simulink model "adc_5g_e2v"  (R2018a)
settings: Solver=VariableStepAuto  StartTime=0.0  StopTime=10.0  RelTol=1e-3
libraries: xbsIndex_r4 x68
settings Model: Creator=jkocz  LastModifiedBy=jackh
settings CodeAppCC: StateflowObjectComments=on

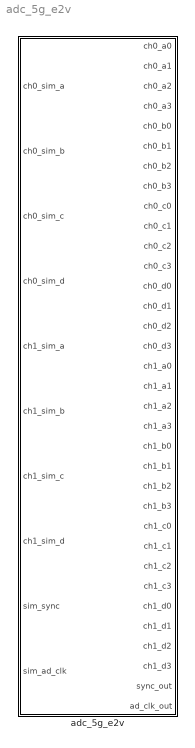
== system adc_5g_e2v ==
  adc_5g_e2v : Subsystem  Tag=xps:adc_5g_e2v  mask(E2V_5g_adc){adc_mode=4-Channel, output_mode=normal mode, chips_num=2, adc_loc=FMC1, f_sample=1000}
      mask prompts: adc_mode "ADC Work mode"; output_mode "ADC Output mode"; chips_num "Number of ADC chips"; adc_loc "ADC board location"; f_sample "ADC Clock Rate(Mhz)"
      mask init:
      | adc_5g_e2v_init(gcb,...
      |     'adc_mode', adc_mode,...
      |     'chips_num',chips_num,...
      |     'adc_loc',adc_loc,...
      |     'f_sample',f_sample);
      mask TypeOptions adc_mode: 1-Channel | 2-Channel | 4-Channel
      mask TypeOptions output_mode: normal mode | test mode
      mask TypeOptions chips_num: 1 | 2
      mask TypeOptions adc_loc: FMC1 | FMC2

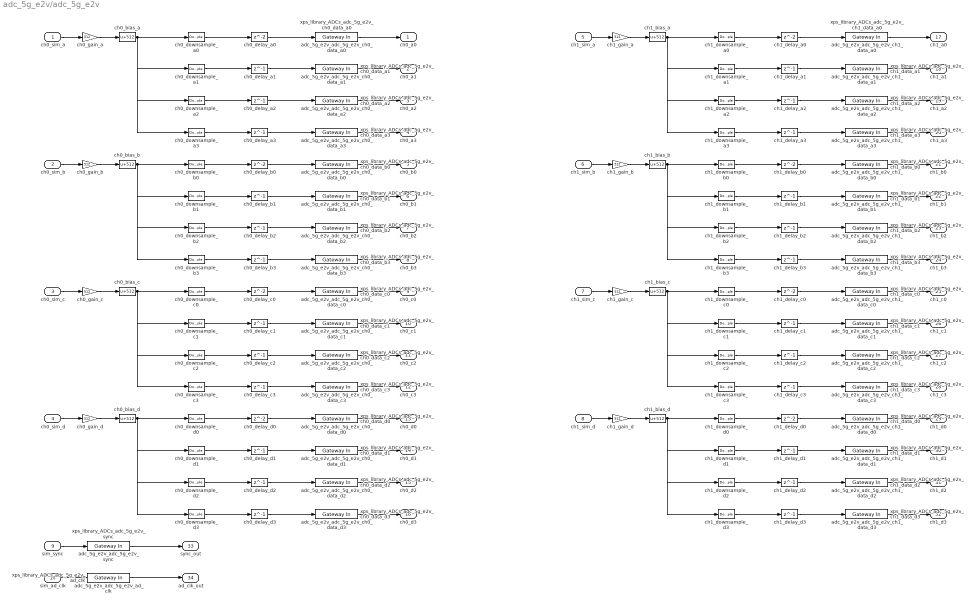
== system adc_5g_e2v/adc_5g_e2v ==
  ch0_sim_a : Inport
  ch0_sim_b : Inport  Port=2
  ch0_sim_c : Inport  Port=3
  ch0_sim_d : Inport  Port=4
  ch1_sim_a : Inport  Port=5
  ch1_sim_b : Inport  Port=6
  ch1_sim_c : Inport  Port=7
  ch1_sim_d : Inport  Port=8
  sim_sync : Inport  Port=9
  sim_ad_clk : Inport  Port=10
  adc_5g_e2v_adc_5g_e2v_ad_clk : xbsIndex_r4/Gateway In  gui_display_data_type=Fixed-point  arith_type=Boolean  n_bits=16  bin_pt=14  preci_type=Single  exp_width=8  frac_width=24  rows=1  columns=1  quantization="Round  (unbiased: +/- Inf)"  overflow=Saturate  period=1  UseAsADC=off  ADCChannel='1'  interface=None  automatic_assignment=on  address_offset=hex2dec('00')  intf_name=''  intf_description=''  default_value=0  timing_constraint=None  locs_specified=off  LOCs={}  io_standard={}  inherit_from_input=off  hdl_port=on  dbl_ovrd=off  block_type=gatewayin
  adc_5g_e2v_adc_5g_e2v_ch0_data_a{0..3} (4 alike) : xbsIndex_r4/Gateway In  gui_display_data_type=Fixed-point  arith_type=Unsigned  n_bits=10  bin_pt=0  preci_type=Single  exp_width=8  frac_width=24  rows=1  columns=1  quantization=Truncate  overflow=Wrap  period=1  UseAsADC=off  ADCChannel='1'  interface=None  automatic_assignment=on  address_offset=hex2dec('00')  intf_name=''  intf_description=''  default_value=0  timing_constraint=None  locs_specified=off  LOCs={}  io_standard={}  inherit_from_input=off  hdl_port=on  dbl_ovrd=off  block_type=gatewayin
  adc_5g_e2v_adc_5g_e2v_ch0_data_b{0..3} (4 alike) : xbsIndex_r4/Gateway In  gui_display_data_type=Fixed-point  arith_type=Unsigned  n_bits=10  bin_pt=0  preci_type=Single  exp_width=8  frac_width=24  rows=1  columns=1  quantization=Truncate  overflow=Wrap  period=1  UseAsADC=off  ADCChannel='1'  interface=None  automatic_assignment=on  address_offset=hex2dec('00')  intf_name=''  intf_description=''  default_value=0  timing_constraint=None  locs_specified=off  LOCs={}  io_standard={}  inherit_from_input=off  hdl_port=on  dbl_ovrd=off  block_type=gatewayin
  adc_5g_e2v_adc_5g_e2v_ch0_data_c{0..3} (4 alike) : xbsIndex_r4/Gateway In  gui_display_data_type=Fixed-point  arith_type=Unsigned  n_bits=10  bin_pt=0  preci_type=Single  exp_width=8  frac_width=24  rows=1  columns=1  quantization=Truncate  overflow=Wrap  period=1  UseAsADC=off  ADCChannel='1'  interface=None  automatic_assignment=on  address_offset=hex2dec('00')  intf_name=''  intf_description=''  default_value=0  timing_constraint=None  locs_specified=off  LOCs={}  io_standard={}  inherit_from_input=off  hdl_port=on  dbl_ovrd=off  block_type=gatewayin
  adc_5g_e2v_adc_5g_e2v_ch0_data_d{0..3} (4 alike) : xbsIndex_r4/Gateway In  gui_display_data_type=Fixed-point  arith_type=Unsigned  n_bits=10  bin_pt=0  preci_type=Single  exp_width=8  frac_width=24  rows=1  columns=1  quantization=Truncate  overflow=Wrap  period=1  UseAsADC=off  ADCChannel='1'  interface=None  automatic_assignment=on  address_offset=hex2dec('00')  intf_name=''  intf_description=''  default_value=0  timing_constraint=None  locs_specified=off  LOCs={}  io_standard={}  inherit_from_input=off  hdl_port=on  dbl_ovrd=off  block_type=gatewayin
  adc_5g_e2v_adc_5g_e2v_ch1_data_a{0..3} (4 alike) : xbsIndex_r4/Gateway In  gui_display_data_type=Fixed-point  arith_type=Unsigned  n_bits=10  bin_pt=0  preci_type=Single  exp_width=8  frac_width=24  rows=1  columns=1  quantization=Truncate  overflow=Wrap  period=1  UseAsADC=off  ADCChannel='1'  interface=None  automatic_assignment=on  address_offset=hex2dec('00')  intf_name=''  intf_description=''  default_value=0  timing_constraint=None  locs_specified=off  LOCs={}  io_standard={}  inherit_from_input=off  hdl_port=on  dbl_ovrd=off  block_type=gatewayin
  adc_5g_e2v_adc_5g_e2v_ch1_data_b{0..3} (4 alike) : xbsIndex_r4/Gateway In  gui_display_data_type=Fixed-point  arith_type=Unsigned  n_bits=10  bin_pt=0  preci_type=Single  exp_width=8  frac_width=24  rows=1  columns=1  quantization=Truncate  overflow=Wrap  period=1  UseAsADC=off  ADCChannel='1'  interface=None  automatic_assignment=on  address_offset=hex2dec('00')  intf_name=''  intf_description=''  default_value=0  timing_constraint=None  locs_specified=off  LOCs={}  io_standard={}  inherit_from_input=off  hdl_port=on  dbl_ovrd=off  block_type=gatewayin
  adc_5g_e2v_adc_5g_e2v_ch1_data_c{0..3} (4 alike) : xbsIndex_r4/Gateway In  gui_display_data_type=Fixed-point  arith_type=Unsigned  n_bits=10  bin_pt=0  preci_type=Single  exp_width=8  frac_width=24  rows=1  columns=1  quantization=Truncate  overflow=Wrap  period=1  UseAsADC=off  ADCChannel='1'  interface=None  automatic_assignment=on  address_offset=hex2dec('00')  intf_name=''  intf_description=''  default_value=0  timing_constraint=None  locs_specified=off  LOCs={}  io_standard={}  inherit_from_input=off  hdl_port=on  dbl_ovrd=off  block_type=gatewayin
  adc_5g_e2v_adc_5g_e2v_ch1_data_d{0..3} (4 alike) : xbsIndex_r4/Gateway In  gui_display_data_type=Fixed-point  arith_type=Unsigned  n_bits=10  bin_pt=0  preci_type=Single  exp_width=8  frac_width=24  rows=1  columns=1  quantization=Truncate  overflow=Wrap  period=1  UseAsADC=off  ADCChannel='1'  interface=None  automatic_assignment=on  address_offset=hex2dec('00')  intf_name=''  intf_description=''  default_value=0  timing_constraint=None  locs_specified=off  LOCs={}  io_standard={}  inherit_from_input=off  hdl_port=on  dbl_ovrd=off  block_type=gatewayin
  adc_5g_e2v_adc_5g_e2v_sync : xbsIndex_r4/Gateway In  gui_display_data_type=Fixed-point  arith_type=Boolean  n_bits=16  bin_pt=14  preci_type=Single  exp_width=8  frac_width=24  rows=1  columns=1  quantization="Round  (unbiased: +/- Inf)"  overflow=Saturate  period=1  UseAsADC=off  ADCChannel='1'  interface=None  automatic_assignment=on  address_offset=hex2dec('00')  intf_name=''  intf_description=''  default_value=0  timing_constraint=None  locs_specified=off  LOCs={}  io_standard={}  inherit_from_input=off  hdl_port=on  dbl_ovrd=off  block_type=gatewayin
  ch0_bias_a : Bias  Bias=512  SaturateOnIntegerOverflow=on
  ch0_bias_b : Bias  Bias=512  SaturateOnIntegerOverflow=on
  ch0_bias_c : Bias  Bias=512  SaturateOnIntegerOverflow=on
  ch0_bias_d : Bias  Bias=512  SaturateOnIntegerOverflow=on
  ch0_delay_a0 : Delay  InitialCondition=0  InputProcessing=Inherited
  ch0_delay_a1 : Delay  DelayLength=1  InitialCondition=0  InputProcessing=Inherited
  ch0_delay_a2 : Delay  DelayLength=1  InitialCondition=0  InputProcessing=Inherited
  ch0_delay_a3 : Delay  DelayLength=1  InitialCondition=0  InputProcessing=Inherited
  ch0_delay_b0 : Delay  InitialCondition=0  InputProcessing=Inherited
  ch0_delay_b1 : Delay  DelayLength=1  InitialCondition=0  InputProcessing=Inherited
  ch0_delay_b2 : Delay  DelayLength=1  InitialCondition=0  InputProcessing=Inherited
  ch0_delay_b3 : Delay  DelayLength=1  InitialCondition=0  InputProcessing=Inherited
  ch0_delay_c0 : Delay  InitialCondition=0  InputProcessing=Inherited
  ch0_delay_c1 : Delay  DelayLength=1  InitialCondition=0  InputProcessing=Inherited
  ch0_delay_c2 : Delay  DelayLength=1  InitialCondition=0  InputProcessing=Inherited
  ch0_delay_c3 : Delay  DelayLength=1  InitialCondition=0  InputProcessing=Inherited
  ch0_delay_d0 : Delay  InitialCondition=0  InputProcessing=Inherited
  ch0_delay_d1 : Delay  DelayLength=1  InitialCondition=0  InputProcessing=Inherited
  ch0_delay_d2 : Delay  DelayLength=1  InitialCondition=0  InputProcessing=Inherited
  ch0_delay_d3 : Delay  DelayLength=1  InitialCondition=0  InputProcessing=Inherited
  ch0_downsample_a0 : DownSample  N=4  RateOptions=Allow multirate processing
  ch0_downsample_a1 : DownSample  N=4  phase=1  RateOptions=Allow multirate processing
  ch0_downsample_a2 : DownSample  N=4  phase=2  RateOptions=Allow multirate processing
  ch0_downsample_a3 : DownSample  N=4  phase=3  RateOptions=Allow multirate processing
  ch0_downsample_b0 : DownSample  N=4  RateOptions=Allow multirate processing
  ch0_downsample_b1 : DownSample  N=4  phase=1  RateOptions=Allow multirate processing
  ch0_downsample_b2 : DownSample  N=4  phase=2  RateOptions=Allow multirate processing
  ch0_downsample_b3 : DownSample  N=4  phase=3  RateOptions=Allow multirate processing
  ch0_downsample_c0 : DownSample  N=4  RateOptions=Allow multirate processing
  ch0_downsample_c1 : DownSample  N=4  phase=1  RateOptions=Allow multirate processing
  ch0_downsample_c2 : DownSample  N=4  phase=2  RateOptions=Allow multirate processing
  ch0_downsample_c3 : DownSample  N=4  phase=3  RateOptions=Allow multirate processing
  ch0_downsample_d0 : DownSample  N=4  RateOptions=Allow multirate processing
  ch0_downsample_d1 : DownSample  N=4  phase=1  RateOptions=Allow multirate processing
  ch0_downsample_d2 : DownSample  N=4  phase=2  RateOptions=Allow multirate processing
  ch0_downsample_d3 : DownSample  N=4  phase=3  RateOptions=Allow multirate processing
  ch0_gain_a : Gain  Gain=512  SaturateOnIntegerOverflow=on  OutDataTypeStr=Inherit: Same as input  ParamDataTypeStr=Inherit: Same as input
  ch0_gain_b : Gain  Gain=512  SaturateOnIntegerOverflow=on  OutDataTypeStr=Inherit: Same as input  ParamDataTypeStr=Inherit: Same as input
  ch0_gain_c : Gain  Gain=512  SaturateOnIntegerOverflow=on  OutDataTypeStr=Inherit: Same as input  ParamDataTypeStr=Inherit: Same as input
  ch0_gain_d : Gain  Gain=512  SaturateOnIntegerOverflow=on  OutDataTypeStr=Inherit: Same as input  ParamDataTypeStr=Inherit: Same as input
  ch1_bias_a : Bias  Bias=512  SaturateOnIntegerOverflow=on
  ch1_bias_b : Bias  Bias=512  SaturateOnIntegerOverflow=on
  ch1_bias_c : Bias  Bias=512  SaturateOnIntegerOverflow=on
  ch1_bias_d : Bias  Bias=512  SaturateOnIntegerOverflow=on
  ch1_delay_a0 : Delay  InitialCondition=0  InputProcessing=Inherited
  ch1_delay_a1 : Delay  DelayLength=1  InitialCondition=0  InputProcessing=Inherited
  ch1_delay_a2 : Delay  DelayLength=1  InitialCondition=0  InputProcessing=Inherited
  ch1_delay_a3 : Delay  DelayLength=1  InitialCondition=0  InputProcessing=Inherited
  ch1_delay_b0 : Delay  InitialCondition=0  InputProcessing=Inherited
  ch1_delay_b1 : Delay  DelayLength=1  InitialCondition=0  InputProcessing=Inherited
  ch1_delay_b2 : Delay  DelayLength=1  InitialCondition=0  InputProcessing=Inherited
  ch1_delay_b3 : Delay  DelayLength=1  InitialCondition=0  InputProcessing=Inherited
  ch1_delay_c0 : Delay  InitialCondition=0  InputProcessing=Inherited
  ch1_delay_c1 : Delay  DelayLength=1  InitialCondition=0  InputProcessing=Inherited
  ch1_delay_c2 : Delay  DelayLength=1  InitialCondition=0  InputProcessing=Inherited
  ch1_delay_c3 : Delay  DelayLength=1  InitialCondition=0  InputProcessing=Inherited
  ch1_delay_d0 : Delay  InitialCondition=0  InputProcessing=Inherited
  ch1_delay_d1 : Delay  DelayLength=1  InitialCondition=0  InputProcessing=Inherited
  ch1_delay_d2 : Delay  DelayLength=1  InitialCondition=0  InputProcessing=Inherited
  ch1_delay_d3 : Delay  DelayLength=1  InitialCondition=0  InputProcessing=Inherited
  ch1_downsample_a0 : DownSample  N=4  RateOptions=Allow multirate processing
  ch1_downsample_a1 : DownSample  N=4  phase=1  RateOptions=Allow multirate processing
  ch1_downsample_a2 : DownSample  N=4  phase=2  RateOptions=Allow multirate processing
  ch1_downsample_a3 : DownSample  N=4  phase=3  RateOptions=Allow multirate processing
  ch1_downsample_b0 : DownSample  N=4  RateOptions=Allow multirate processing
  ch1_downsample_b1 : DownSample  N=4  phase=1  RateOptions=Allow multirate processing
  ch1_downsample_b2 : DownSample  N=4  phase=2  RateOptions=Allow multirate processing
  ch1_downsample_b3 : DownSample  N=4  phase=3  RateOptions=Allow multirate processing
  ch1_downsample_c0 : DownSample  N=4  RateOptions=Allow multirate processing
  ch1_downsample_c1 : DownSample  N=4  phase=1  RateOptions=Allow multirate processing
  ch1_downsample_c2 : DownSample  N=4  phase=2  RateOptions=Allow multirate processing
  ch1_downsample_c3 : DownSample  N=4  phase=3  RateOptions=Allow multirate processing
  ch1_downsample_d0 : DownSample  N=4  RateOptions=Allow multirate processing
  ch1_downsample_d1 : DownSample  N=4  phase=1  RateOptions=Allow multirate processing
  ch1_downsample_d2 : DownSample  N=4  phase=2  RateOptions=Allow multirate processing
  ch1_downsample_d3 : DownSample  N=4  phase=3  RateOptions=Allow multirate processing
  ch1_gain_a : Gain  Gain=512  SaturateOnIntegerOverflow=on  OutDataTypeStr=Inherit: Same as input  ParamDataTypeStr=Inherit: Same as input
  ch1_gain_b : Gain  Gain=512  SaturateOnIntegerOverflow=on  OutDataTypeStr=Inherit: Same as input  ParamDataTypeStr=Inherit: Same as input
  ch1_gain_c : Gain  Gain=512  SaturateOnIntegerOverflow=on  OutDataTypeStr=Inherit: Same as input  ParamDataTypeStr=Inherit: Same as input
  ch1_gain_d : Gain  Gain=512  SaturateOnIntegerOverflow=on  OutDataTypeStr=Inherit: Same as input  ParamDataTypeStr=Inherit: Same as input
  xps_library_ADCs_adc_5g_e2v_ad_clk : xbsIndex_r4/Gateway In  gui_display_data_type=Fixed-point  arith_type=Boolean  n_bits=16  bin_pt=14  preci_type=Single  exp_width=8  frac_width=24  rows=1  columns=1  quantization="Round  (unbiased: +/- Inf)"  overflow=Saturate  period=1  UseAsADC=off  ADCChannel='1'  interface=None  automatic_assignment=on  address_offset=hex2dec('00')  intf_name=''  intf_description=''  default_value=0  timing_constraint=None  locs_specified=off  LOCs={}  io_standard={}  inherit_from_input=off  hdl_port=on  dbl_ovrd=off  block_type=gatewayin
  xps_library_ADCs_adc_5g_e2v_ch0_data_a{0..3} (4 alike) : xbsIndex_r4/Gateway In  gui_display_data_type=Fixed-point  arith_type=Unsigned  n_bits=10  bin_pt=0  preci_type=Single  exp_width=8  frac_width=24  rows=1  columns=1  quantization=Truncate  overflow=Wrap  period=1  UseAsADC=off  ADCChannel='1'  interface=None  automatic_assignment=on  address_offset=hex2dec('00')  intf_name=''  intf_description=''  default_value=0  timing_constraint=None  locs_specified=off  LOCs={}  io_standard={}  inherit_from_input=off  hdl_port=on  dbl_ovrd=off  block_type=gatewayin
  xps_library_ADCs_adc_5g_e2v_ch0_data_b{0..3} (4 alike) : xbsIndex_r4/Gateway In  gui_display_data_type=Fixed-point  arith_type=Unsigned  n_bits=10  bin_pt=0  preci_type=Single  exp_width=8  frac_width=24  rows=1  columns=1  quantization=Truncate  overflow=Wrap  period=1  UseAsADC=off  ADCChannel='1'  interface=None  automatic_assignment=on  address_offset=hex2dec('00')  intf_name=''  intf_description=''  default_value=0  timing_constraint=None  locs_specified=off  LOCs={}  io_standard={}  inherit_from_input=off  hdl_port=on  dbl_ovrd=off  block_type=gatewayin
  xps_library_ADCs_adc_5g_e2v_ch0_data_c{0..3} (4 alike) : xbsIndex_r4/Gateway In  gui_display_data_type=Fixed-point  arith_type=Unsigned  n_bits=10  bin_pt=0  preci_type=Single  exp_width=8  frac_width=24  rows=1  columns=1  quantization=Truncate  overflow=Wrap  period=1  UseAsADC=off  ADCChannel='1'  interface=None  automatic_assignment=on  address_offset=hex2dec('00')  intf_name=''  intf_description=''  default_value=0  timing_constraint=None  locs_specified=off  LOCs={}  io_standard={}  inherit_from_input=off  hdl_port=on  dbl_ovrd=off  block_type=gatewayin
  xps_library_ADCs_adc_5g_e2v_ch0_data_d{0..3} (4 alike) : xbsIndex_r4/Gateway In  gui_display_data_type=Fixed-point  arith_type=Unsigned  n_bits=10  bin_pt=0  preci_type=Single  exp_width=8  frac_width=24  rows=1  columns=1  quantization=Truncate  overflow=Wrap  period=1  UseAsADC=off  ADCChannel='1'  interface=None  automatic_assignment=on  address_offset=hex2dec('00')  intf_name=''  intf_description=''  default_value=0  timing_constraint=None  locs_specified=off  LOCs={}  io_standard={}  inherit_from_input=off  hdl_port=on  dbl_ovrd=off  block_type=gatewayin
  xps_library_ADCs_adc_5g_e2v_ch1_data_a{0..3} (4 alike) : xbsIndex_r4/Gateway In  gui_display_data_type=Fixed-point  arith_type=Unsigned  n_bits=10  bin_pt=0  preci_type=Single  exp_width=8  frac_width=24  rows=1  columns=1  quantization=Truncate  overflow=Wrap  period=1  UseAsADC=off  ADCChannel='1'  interface=None  automatic_assignment=on  address_offset=hex2dec('00')  intf_name=''  intf_description=''  default_value=0  timing_constraint=None  locs_specified=off  LOCs={}  io_standard={}  inherit_from_input=off  hdl_port=on  dbl_ovrd=off  block_type=gatewayin
  xps_library_ADCs_adc_5g_e2v_ch1_data_b{0..3} (4 alike) : xbsIndex_r4/Gateway In  gui_display_data_type=Fixed-point  arith_type=Unsigned  n_bits=10  bin_pt=0  preci_type=Single  exp_width=8  frac_width=24  rows=1  columns=1  quantization=Truncate  overflow=Wrap  period=1  UseAsADC=off  ADCChannel='1'  interface=None  automatic_assignment=on  address_offset=hex2dec('00')  intf_name=''  intf_description=''  default_value=0  timing_constraint=None  locs_specified=off  LOCs={}  io_standard={}  inherit_from_input=off  hdl_port=on  dbl_ovrd=off  block_type=gatewayin
  xps_library_ADCs_adc_5g_e2v_ch1_data_c{0..3} (4 alike) : xbsIndex_r4/Gateway In  gui_display_data_type=Fixed-point  arith_type=Unsigned  n_bits=10  bin_pt=0  preci_type=Single  exp_width=8  frac_width=24  rows=1  columns=1  quantization=Truncate  overflow=Wrap  period=1  UseAsADC=off  ADCChannel='1'  interface=None  automatic_assignment=on  address_offset=hex2dec('00')  intf_name=''  intf_description=''  default_value=0  timing_constraint=None  locs_specified=off  LOCs={}  io_standard={}  inherit_from_input=off  hdl_port=on  dbl_ovrd=off  block_type=gatewayin
  xps_library_ADCs_adc_5g_e2v_ch1_data_d{0..3} (4 alike) : xbsIndex_r4/Gateway In  gui_display_data_type=Fixed-point  arith_type=Unsigned  n_bits=10  bin_pt=0  preci_type=Single  exp_width=8  frac_width=24  rows=1  columns=1  quantization=Truncate  overflow=Wrap  period=1  UseAsADC=off  ADCChannel='1'  interface=None  automatic_assignment=on  address_offset=hex2dec('00')  intf_name=''  intf_description=''  default_value=0  timing_constraint=None  locs_specified=off  LOCs={}  io_standard={}  inherit_from_input=off  hdl_port=on  dbl_ovrd=off  block_type=gatewayin
  xps_library_ADCs_adc_5g_e2v_sync : xbsIndex_r4/Gateway In  gui_display_data_type=Fixed-point  arith_type=Boolean  n_bits=16  bin_pt=14  preci_type=Single  exp_width=8  frac_width=24  rows=1  columns=1  quantization="Round  (unbiased: +/- Inf)"  overflow=Saturate  period=1  UseAsADC=off  ADCChannel='1'  interface=None  automatic_assignment=on  address_offset=hex2dec('00')  intf_name=''  intf_description=''  default_value=0  timing_constraint=None  locs_specified=off  LOCs={}  io_standard={}  inherit_from_input=off  hdl_port=on  dbl_ovrd=off  block_type=gatewayin
  ch0_a0 : Outport
  ch0_a1 : Outport  Port=2
  ch0_a2 : Outport  Port=3
  ch0_a3 : Outport  Port=4
  ch0_b0 : Outport  Port=5
  ch0_b1 : Outport  Port=6
  ch0_b2 : Outport  Port=7
  ch0_b3 : Outport  Port=8
  ch0_c0 : Outport  Port=9
  ch0_c1 : Outport  Port=10
  ch0_c2 : Outport  Port=11
  ch0_c3 : Outport  Port=12
  ch0_d0 : Outport  Port=13
  ch0_d1 : Outport  Port=14
  ch0_d2 : Outport  Port=15
  ch0_d3 : Outport  Port=16
  ch1_a0 : Outport  Port=17
  ch1_a1 : Outport  Port=18
  ch1_a2 : Outport  Port=19
  ch1_a3 : Outport  Port=20
  ch1_b0 : Outport  Port=21
  ch1_b1 : Outport  Port=22
  ch1_b2 : Outport  Port=23
  ch1_b3 : Outport  Port=24
  ch1_c0 : Outport  Port=25
  ch1_c1 : Outport  Port=26
  ch1_c2 : Outport  Port=27
  ch1_c3 : Outport  Port=28
  ch1_d0 : Outport  Port=29
  ch1_d1 : Outport  Port=30
  ch1_d2 : Outport  Port=31
  ch1_d3 : Outport  Port=32
  sync_out : Outport  Port=33
  ad_clk_out : Outport  Port=34
  wires:
  ch0_sim_a/1 -> ch0_gain_a/1
  ch0_gain_a/1 -> ch0_bias_a/1
  ch0_bias_a/1 -> ch0_downsample_a0/1, ch0_downsample_a1/1, ch0_downsample_a2/1, ch0_downsample_a3/1
  ch0_downsample_a0/1 -> ch0_delay_a0/1
  ch0_delay_a0/1 -> adc_5g_e2v_adc_5g_e2v_ch0_data_a0/1
  adc_5g_e2v_adc_5g_e2v_ch0_data_a0/1 -> ch0_a0/1
  ch0_downsample_a1/1 -> ch0_delay_a1/1
  ch0_delay_a1/1 -> adc_5g_e2v_adc_5g_e2v_ch0_data_a1/1
  adc_5g_e2v_adc_5g_e2v_ch0_data_a1/1 -> ch0_a1/1
  ch0_downsample_a2/1 -> ch0_delay_a2/1
  ch0_delay_a2/1 -> adc_5g_e2v_adc_5g_e2v_ch0_data_a2/1
  adc_5g_e2v_adc_5g_e2v_ch0_data_a2/1 -> ch0_a2/1
  ch0_downsample_a3/1 -> ch0_delay_a3/1
  ch0_delay_a3/1 -> adc_5g_e2v_adc_5g_e2v_ch0_data_a3/1
  adc_5g_e2v_adc_5g_e2v_ch0_data_a3/1 -> ch0_a3/1
  ch0_sim_b/1 -> ch0_gain_b/1
  ch0_gain_b/1 -> ch0_bias_b/1
  ch0_bias_b/1 -> ch0_downsample_b0/1, ch0_downsample_b1/1, ch0_downsample_b2/1, ch0_downsample_b3/1
  ch0_downsample_b0/1 -> ch0_delay_b0/1
  ch0_delay_b0/1 -> adc_5g_e2v_adc_5g_e2v_ch0_data_b0/1
  adc_5g_e2v_adc_5g_e2v_ch0_data_b0/1 -> ch0_b0/1
  ch0_downsample_b1/1 -> ch0_delay_b1/1
  ch0_delay_b1/1 -> adc_5g_e2v_adc_5g_e2v_ch0_data_b1/1
  adc_5g_e2v_adc_5g_e2v_ch0_data_b1/1 -> ch0_b1/1
  ch0_downsample_b2/1 -> ch0_delay_b2/1
  ch0_delay_b2/1 -> adc_5g_e2v_adc_5g_e2v_ch0_data_b2/1
  adc_5g_e2v_adc_5g_e2v_ch0_data_b2/1 -> ch0_b2/1
  ch0_downsample_b3/1 -> ch0_delay_b3/1
  ch0_delay_b3/1 -> adc_5g_e2v_adc_5g_e2v_ch0_data_b3/1
  adc_5g_e2v_adc_5g_e2v_ch0_data_b3/1 -> ch0_b3/1
  ch0_sim_c/1 -> ch0_gain_c/1
  ch0_gain_c/1 -> ch0_bias_c/1
  ch0_bias_c/1 -> ch0_downsample_c0/1, ch0_downsample_c1/1, ch0_downsample_c2/1, ch0_downsample_c3/1
  ch0_downsample_c0/1 -> ch0_delay_c0/1
  ch0_delay_c0/1 -> adc_5g_e2v_adc_5g_e2v_ch0_data_c0/1
  adc_5g_e2v_adc_5g_e2v_ch0_data_c0/1 -> ch0_c0/1
  ch0_downsample_c1/1 -> ch0_delay_c1/1
  ch0_delay_c1/1 -> adc_5g_e2v_adc_5g_e2v_ch0_data_c1/1
  adc_5g_e2v_adc_5g_e2v_ch0_data_c1/1 -> ch0_c1/1
  ch0_downsample_c2/1 -> ch0_delay_c2/1
  ch0_delay_c2/1 -> adc_5g_e2v_adc_5g_e2v_ch0_data_c2/1
  adc_5g_e2v_adc_5g_e2v_ch0_data_c2/1 -> ch0_c2/1
  ch0_downsample_c3/1 -> ch0_delay_c3/1
  ch0_delay_c3/1 -> adc_5g_e2v_adc_5g_e2v_ch0_data_c3/1
  adc_5g_e2v_adc_5g_e2v_ch0_data_c3/1 -> ch0_c3/1
  ch0_sim_d/1 -> ch0_gain_d/1
  ch0_gain_d/1 -> ch0_bias_d/1
  ch0_bias_d/1 -> ch0_downsample_d0/1, ch0_downsample_d1/1, ch0_downsample_d2/1, ch0_downsample_d3/1
  ch0_downsample_d0/1 -> ch0_delay_d0/1
  ch0_delay_d0/1 -> adc_5g_e2v_adc_5g_e2v_ch0_data_d0/1
  adc_5g_e2v_adc_5g_e2v_ch0_data_d0/1 -> ch0_d0/1
  ch0_downsample_d1/1 -> ch0_delay_d1/1
  ch0_delay_d1/1 -> adc_5g_e2v_adc_5g_e2v_ch0_data_d1/1
  adc_5g_e2v_adc_5g_e2v_ch0_data_d1/1 -> ch0_d1/1
  ch0_downsample_d2/1 -> ch0_delay_d2/1
  ch0_delay_d2/1 -> adc_5g_e2v_adc_5g_e2v_ch0_data_d2/1
  adc_5g_e2v_adc_5g_e2v_ch0_data_d2/1 -> ch0_d2/1
  ch0_downsample_d3/1 -> ch0_delay_d3/1
  ch0_delay_d3/1 -> adc_5g_e2v_adc_5g_e2v_ch0_data_d3/1
  adc_5g_e2v_adc_5g_e2v_ch0_data_d3/1 -> ch0_d3/1
  ch1_sim_a/1 -> ch1_gain_a/1
  ch1_gain_a/1 -> ch1_bias_a/1
  ch1_bias_a/1 -> ch1_downsample_a0/1, ch1_downsample_a1/1, ch1_downsample_a2/1, ch1_downsample_a3/1
  ch1_downsample_a0/1 -> ch1_delay_a0/1
  ch1_delay_a0/1 -> adc_5g_e2v_adc_5g_e2v_ch1_data_a0/1
  adc_5g_e2v_adc_5g_e2v_ch1_data_a0/1 -> ch1_a0/1
  ch1_downsample_a1/1 -> ch1_delay_a1/1
  ch1_delay_a1/1 -> adc_5g_e2v_adc_5g_e2v_ch1_data_a1/1
  adc_5g_e2v_adc_5g_e2v_ch1_data_a1/1 -> ch1_a1/1
  ch1_downsample_a2/1 -> ch1_delay_a2/1
  ch1_delay_a2/1 -> adc_5g_e2v_adc_5g_e2v_ch1_data_a2/1
  adc_5g_e2v_adc_5g_e2v_ch1_data_a2/1 -> ch1_a2/1
  ch1_downsample_a3/1 -> ch1_delay_a3/1
  ch1_delay_a3/1 -> adc_5g_e2v_adc_5g_e2v_ch1_data_a3/1
  adc_5g_e2v_adc_5g_e2v_ch1_data_a3/1 -> ch1_a3/1
  ch1_sim_b/1 -> ch1_gain_b/1
  ch1_gain_b/1 -> ch1_bias_b/1
  ch1_bias_b/1 -> ch1_downsample_b0/1, ch1_downsample_b1/1, ch1_downsample_b2/1, ch1_downsample_b3/1
  ch1_downsample_b0/1 -> ch1_delay_b0/1
  ch1_delay_b0/1 -> adc_5g_e2v_adc_5g_e2v_ch1_data_b0/1
  adc_5g_e2v_adc_5g_e2v_ch1_data_b0/1 -> ch1_b0/1
  ch1_downsample_b1/1 -> ch1_delay_b1/1
  ch1_delay_b1/1 -> adc_5g_e2v_adc_5g_e2v_ch1_data_b1/1
  adc_5g_e2v_adc_5g_e2v_ch1_data_b1/1 -> ch1_b1/1
  ch1_downsample_b2/1 -> ch1_delay_b2/1
  ch1_delay_b2/1 -> adc_5g_e2v_adc_5g_e2v_ch1_data_b2/1
  adc_5g_e2v_adc_5g_e2v_ch1_data_b2/1 -> ch1_b2/1
  ch1_downsample_b3/1 -> ch1_delay_b3/1
  ch1_delay_b3/1 -> adc_5g_e2v_adc_5g_e2v_ch1_data_b3/1
  adc_5g_e2v_adc_5g_e2v_ch1_data_b3/1 -> ch1_b3/1
  ch1_sim_c/1 -> ch1_gain_c/1
  ch1_gain_c/1 -> ch1_bias_c/1
  ch1_bias_c/1 -> ch1_downsample_c0/1, ch1_downsample_c1/1, ch1_downsample_c2/1, ch1_downsample_c3/1
  ch1_downsample_c0/1 -> ch1_delay_c0/1
  ch1_delay_c0/1 -> adc_5g_e2v_adc_5g_e2v_ch1_data_c0/1
  adc_5g_e2v_adc_5g_e2v_ch1_data_c0/1 -> ch1_c0/1
  ch1_downsample_c1/1 -> ch1_delay_c1/1
  ch1_delay_c1/1 -> adc_5g_e2v_adc_5g_e2v_ch1_data_c1/1
  adc_5g_e2v_adc_5g_e2v_ch1_data_c1/1 -> ch1_c1/1
  ch1_downsample_c2/1 -> ch1_delay_c2/1
  ch1_delay_c2/1 -> adc_5g_e2v_adc_5g_e2v_ch1_data_c2/1
  adc_5g_e2v_adc_5g_e2v_ch1_data_c2/1 -> ch1_c2/1
  ch1_downsample_c3/1 -> ch1_delay_c3/1
  ch1_delay_c3/1 -> adc_5g_e2v_adc_5g_e2v_ch1_data_c3/1
  adc_5g_e2v_adc_5g_e2v_ch1_data_c3/1 -> ch1_c3/1
  ch1_sim_d/1 -> ch1_gain_d/1
  ch1_gain_d/1 -> ch1_bias_d/1
  ch1_bias_d/1 -> ch1_downsample_d0/1, ch1_downsample_d1/1, ch1_downsample_d2/1, ch1_downsample_d3/1
  ch1_downsample_d0/1 -> ch1_delay_d0/1
  ch1_delay_d0/1 -> adc_5g_e2v_adc_5g_e2v_ch1_data_d0/1
  adc_5g_e2v_adc_5g_e2v_ch1_data_d0/1 -> ch1_d0/1
  ch1_downsample_d1/1 -> ch1_delay_d1/1
  ch1_delay_d1/1 -> adc_5g_e2v_adc_5g_e2v_ch1_data_d1/1
  adc_5g_e2v_adc_5g_e2v_ch1_data_d1/1 -> ch1_d1/1
  ch1_downsample_d2/1 -> ch1_delay_d2/1
  ch1_delay_d2/1 -> adc_5g_e2v_adc_5g_e2v_ch1_data_d2/1
  adc_5g_e2v_adc_5g_e2v_ch1_data_d2/1 -> ch1_d2/1
  ch1_downsample_d3/1 -> ch1_delay_d3/1
  ch1_delay_d3/1 -> adc_5g_e2v_adc_5g_e2v_ch1_data_d3/1
  adc_5g_e2v_adc_5g_e2v_ch1_data_d3/1 -> ch1_d3/1
  sim_sync/1 -> adc_5g_e2v_adc_5g_e2v_sync/1
  adc_5g_e2v_adc_5g_e2v_sync/1 -> sync_out/1
  sim_ad_clk/1 -> adc_5g_e2v_adc_5g_e2v_ad_clk/1
  adc_5g_e2v_adc_5g_e2v_ad_clk/1 -> ad_clk_out/1
